simulink model "Resocharge"  (R2023a)
settings: Solver=ode1  StartTime=0.0  StopTime=.4  FixedStep=2e-7  RelTol=1e-3
undefined symbols (not defined in the file): Ion, Lithium
libraries: spsSeriesRLCBranchLib x6, spsVoltageMeasurementLib x6, spsCurrentMeasurementLib x5, spsDiodeLib x4, spsMosfetLib x4, spsACVoltageSourceLib x1, spsBatteryLib x1, simulink x1, spsMutualInductanceLib x1, spsUniversalBridgeLib x1, spspowerguiLib x1
settings Model: Creator=Harish Kumar M  LastModifiedBy=Harish Kumar M

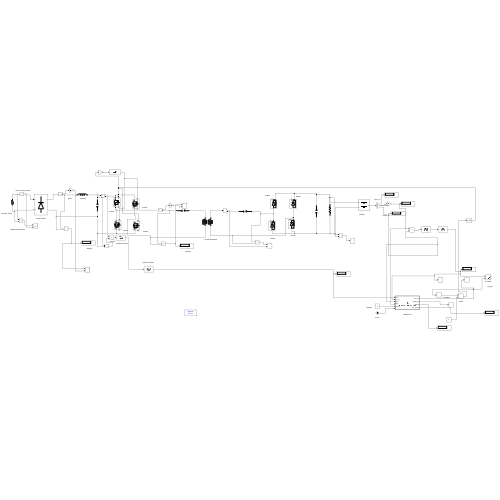
[thumbnail: Simulink's stored preview of the top-level diagram]
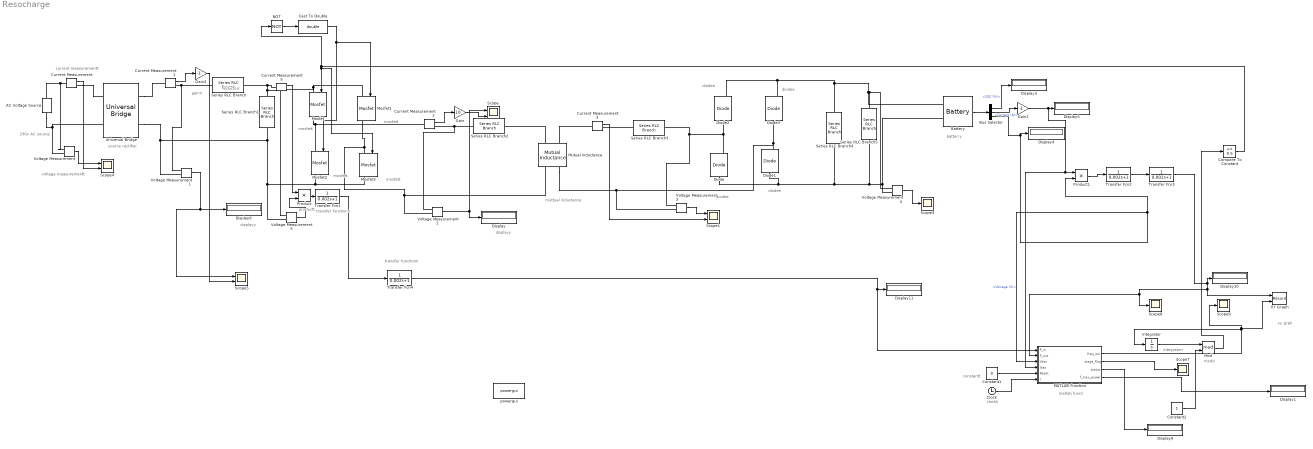
== system Resocharge ==
  note: modd
  note: xy grph
  note: integratorr
  note: constantt
  note: clockk
  note: matlab funcn
  note: batterry
  note: displayy
  note: diodee
  note: muttual inductance
  note: productt
  note: transfer functionn
  note: mosfett
  note: inductorr
  note: gainn
  note: source rectifier
  note: voltage measurementt
  note: 230v AC source
  note: current measurementt
  note: transfer functionn
  note: diodee
  note: diodee
  note: diodee
  note: mosfett
  note: mosfett
  note: mosfett
  note: displayy
  AC Voltage Source : spsACVoltageSourceLib/AC Voltage Source  Amplitude=230*sqrt(2)  Phase=0  Frequency=50  SampleTime=0  Measurements=None  BusType=swing  Pref=10e3  Qref=0  Qmin=-inf  Qmax=+inf
  Battery : spsBatteryLib/Battery  BatType=Lithium-Ion  ShowTempParam=off  ThermalPreset=no  ShowAgeParam=off  NomV=400  NomQ=100  SOC=50  Batt_Tr=1  PresetModel=on  MaxQ=100  MinV=300  FullV=465.5949  Dis_rate=43.4783  R=0.04  Normal_OP=90.4348  expZone="[432.1543      4.913043]"  current=[6.5 13 32.5]  Units=Time  Tci=20  NomT=20  T2=-30  MaxQ2=4.8  FullV2=7.1  Normal_OP2=5.655  expZone2="[6.58           1]"  Rca=0.6  ti=2000  Dp=0  Neq0=0  Tsim=1e6  Ta1=25  Qeol=5.4*0.9  Reol=0.013333*1.2  Char_age=[2.3478, 3]  Dis_age=[2.3478, 10]  N1=1500  N2=10500  N3=1000  N4=1400  Ta2=45  N5=950
  Bus Selector : BusSelector  OutputSignals=SOC (%),Current (A),Voltage (V)
  Cast To Double : DataTypeConversion  OutDataTypeStr=double  SaturateOnIntegerOverflow=off  RndMeth=Floor
  Clock : Clock
  Compare To Constant : simulink/Logic and Bit Operations/Compare To Constant  relop=<=  const=0.5  OutDataTypeStr=boolean
  Constant1 : Constant  Value=0
  Constant2 : Constant
  Current Measurement{,1..3,5} (5 alike) : spsCurrentMeasurementLib/Current Measurement  PhasorSimulation=off  OutputType=Complex  PSBequivalent=0
  Diode{,1..3} (4 alike) : spsDiodeLib/Diode  Ron=0.001  Lon=0  Vf=0.8  IC=0  UseSnubber=0  Rs=500  Cs=250e-9  Measurements=on
  Display{,1,3..6,9..11} (9 alike) : Display
  Gain : Gain  Gain=10
  Gain2 : Gain  Gain=-1
  Gain3 : Gain  Gain=-1
  Integrator : Integrator
  MATLAB Function : MATLAB Function  TreatAsAtomicUnit=on  SystemSampleTime=1e-4
  Mod : Math  Operator=mod
  Mosfet{,1..3} (4 alike) : spsMosfetLib/Mosfet  Ron=0.1  Lon=0  Rd=0.01  Vfd=0  IC=0  Rs=1e5  Cs=inf  Measurements=on
  Mutual Inductance : spsMutualInductanceLib/Mutual Inductance  LConnTagsString=a|b  RConnTagsString=A|B  TypeOfMutual=Two or three windings with equal mutual terms  NumberOfWindings=3  SelfImpedance1=[0.05 110e-06]  SelfImpedance2=[ 0.05 110e-6]  ThreeWindings=off  SelfImpedance3=[ 1.1 1.1e-03]  MutualImpedance=[0 27.5e-06]  InductanceMatrix="[1.0 0.9  0.9 ;  0.9 1.0  0.9;  0.9 0.9 1.0 ] * 1e-3"  ResistanceMatrix="[1.0 0.9  0.9 ;  0.9 1.0  0.9;  0.9 0.9 1.0 ]"  Measurements=None
      settings: LibrarySourceBlock=sps_lib/Passives/Mutual Inductance
  NOT : Logic  Operator=NOT  IconShape=distinctive  AllPortsSameDT=off  OutDataTypeStr=boolean
  Product : Product
  Product1 : Product
  Scope{,1,4..5} (4 alike) : Scope  NumInputPorts=2
  Scope{3,7..9} (4 alike) : Scope
  Series RLC Branch : spsSeriesRLCBranchLib/Series RLC Branch  LConnTagsString=__new0  RConnTagsString=__new0  BranchType=L  Resistance=1  Inductance=5e-3  SetiL0=off  InitialCurrent=0  Capacitance=1e-6  Setx0=off  InitialVoltage=0  Measurements=None
  Series RLC Branch1 : spsSeriesRLCBranchLib/Series RLC Branch  LConnTagsString=__new0  RConnTagsString=__new0  BranchType=C  Resistance=1  Inductance=1e-3  SetiL0=off  InitialCurrent=0  Capacitance=3300e-6  Setx0=off  InitialVoltage=0  Measurements=None
  Series RLC Branch2 : spsSeriesRLCBranchLib/Series RLC Branch  LConnTagsString=__new0  RConnTagsString=__new0  BranchType=C  Resistance=1  Inductance=1e-3  SetiL0=off  InitialCurrent=0  Capacitance=38.8e-9  Setx0=off  InitialVoltage=0  Measurements=None
  Series RLC Branch3 : spsSeriesRLCBranchLib/Series RLC Branch  LConnTagsString=__new0  RConnTagsString=__new0  BranchType=C  Resistance=1  Inductance=1e-3  SetiL0=off  InitialCurrent=0  Capacitance=38.8e-9  Setx0=off  InitialVoltage=0  Measurements=None
  Series RLC Branch4 : spsSeriesRLCBranchLib/Series RLC Branch  LConnTagsString=__new0  RConnTagsString=__new0  BranchType=C  Resistance=1  Inductance=1e-3  SetiL0=off  InitialCurrent=0  Capacitance=100e-6  Setx0=on  InitialVoltage=325  Measurements=None
  Series RLC Branch5 : spsSeriesRLCBranchLib/Series RLC Branch  LConnTagsString=__new0  RConnTagsString=__new0  BranchType=R  Resistance=10000  Inductance=1e-3  SetiL0=off  InitialCurrent=0  Capacitance=1e-6  Setx0=off  InitialVoltage=0  Measurements=None
  Transfer Fcn{1..4} (4 alike) : TransferFcn  Denominator=[0.002 1]
  Universal Bridge : spsUniversalBridgeLib/Universal Bridge  Arms=2  SnubberResistance=1e5  SnubberCapacitance=inf  Device=Diodes  Ron=1e-3  Lon=0  ForwardVoltages="[  0  0  ]"  ForwardVoltage=0  GTOparameters=[ 10e-6 , 20e-6 ]  IGBTparameters=[ 1e-6 , 2e-6 ]  Measurements=None  Measurements_2=None  converterType=Rectifier
  Voltage Measurement{,1..5} (6 alike) : spsVoltageMeasurementLib/Voltage Measurement  PhasorSimulation=off  OutputType=Complex  PSBequivalent=0
  XY Graph : Record  FileSettingsInternal="{\"entries\":[{\"content\":{\"excelSettings\":{\"content\":{},\"type\":\"Streamout.ExcelSettings\"}},\"type\":\"Streamout.FileSettingStorage\",\"uuid\":\"\"}],\"packageUris\":[\"http:\\/\\/schema.mathworks.com\\/mf0\\/streamout_blocks\\/R2020a\"],\"version\":\"1.0\"}"  Layout=[1 1]  SignalsInternal="{\"entries\":[{\"content\":{\"signals\":[{\"content\":{\"blockPath\":[],\"dimensions\":[1],\"domain\":\"\",\"lineColor\":\"#a2142f\",\"plots\":[1],\"port\":1,\"signalID\":17,\"signalName\":\"Transfer Fcn3\"},\"type\":\"RecordBlkView.Signal\",\"uuid\":\"\"},{\"content\":{\"blockPath\":[],\"dimensions\":[1],\"domain\":\"\",\"lineColor\":\"#139fff\",\"plots\":[1],\"port\":2,\"signalID\":20,\"signalName\":\"MATLAB Function:1\"},\"type\":\"RecordBlkView.Signal\",\"uuid\":\"\"}]},\"type\":\"RecordBlkView.InputSignals\",\"uuid\":\"\"}],\"packageUris\":[\"http:\\/\\/schema.mathworks.com\\/mf0\\/streamout_blocks\\/R2020a\"],\"version\":\"1.0\"}"  VisualizationBindings="{\"xyplotplugin\":{\"info\":[{\"series\":[{\"bindingParametersList\":[{\"parameter\":\"X-Axis\",\"signalID\":17,\"signalName\":\"Transfer Fcn3\"},{\"parameter\":\"Y-Axis\",\"signalID\":20,\"signalName\":\"MATLAB Function:1\"}],\"seriesID\":38810}],\"subplotID\":1}]}}"  CompatibilityTag=XY
  powergui : spspowerguiLib/powergui  Priority=1  SimulationMode=Discrete  SampleTime=2e-7  frequency=60  Iterations=50  frequencyindice=50  Pbase=100e6  ErrMax=1e-4  UnitsV=kV  UnitsW=MW  buscounter=0  FunctionMessages=off  echomessages=off  EnableUseOfTLC=off  CurrentSourceSwitches=off  DisableSnubberDevices=off  DisableRonSwitches=off  DisableVfSwitches=off  DisplayEquations=off  AutomaticDiscreteSolvers=off  SolverType=Tustin/Backward Euler (TBE)  Interpol=off  ExternalGateDelay=off  methode=off  Ts=100  x0status=blocks  SPID=on  SwTol=0  HookPort=off  NonlinearTolerance=1e-4  nMaxIteration=100  ContinueOnMaxIteration=off  RestoreLinks=warning  ResistiveCurrentMeasurement=off  Frange=[0:2:500]  Ylog=off  Xlog=on  ShowGrid=off  save=off  variable=ZData  structure=0  ZoomFFT=off  StartTime=0.0  cycles=1  DisplayStyle=1  fundamental=60  FreqAxis=off  MaxFrequency=1000  frequencyindicesteady=1  RmsSteady=1  display=off
  wires:
  NOT/1 -> Cast To Double/1
  Cast To Double/1 -> Mosfet1/1, Mosfet2/1
  Current Measurement2/1 -> Gain/1
  Voltage Measurement2/1 -> Scope/1, Display/1
  Current Measurement3/1 -> Scope1/2
  Voltage Measurement3/1 -> Scope1/1
  Voltage Measurement4/1 -> Scope3/1
  Battery/1 -> Bus Selector/1
  Bus Selector/1 -> Display3/1  "<SOC (%)>"
  Bus Selector/3 -> Product1/2, MATLAB Function/3(Vbat), Display4/1  "<Voltage (V)>"
  Bus Selector/2 -> Gain2/1  "<Current (A)>"
  Current Measurement/1 -> Scope4/2
  Voltage Measurement/1 -> Scope4/1
  Current Measurement1/1 -> Gain3/1
  Gain3/1 -> Scope5/2
  Voltage Measurement1/1 -> Display6/1, Scope5/1
  Gain/1 -> Scope/2
  Current Measurement5/1 -> Product/1
  Voltage Measurement5/1 -> Product/2
  Product/1 -> Transfer Fcn1/1
  Transfer Fcn1/1 -> Transfer Fcn4/1
  Product1/1 -> Transfer Fcn2/1
  Integrator/1 -> Mod/1
  Constant2/1 -> Mod/2
  Mod/1 -> Compare To Constant/1
  Compare To Constant/1 -> NOT/1, Mosfet3/1, Mosfet/1
  MATLAB Function/2(stage_flag) -> Scope7/1
  Transfer Fcn2/1 -> Transfer Fcn3/1
  Transfer Fcn3/1 -> Display10/1, XY Graph/1, MATLAB Function/2(P_out), Scope8/1
  Transfer Fcn4/1 -> MATLAB Function/1(P_in), Display11/1
  MATLAB Function/3(status) -> Display9/1
  Constant1/1 -> MATLAB Function/5(Reset)
  Clock/1 -> MATLAB Function/6(t)
  Gain2/1 -> MATLAB Function/4(Ibat), Product1/1, Display5/1
  MATLAB Function/1(freq_out) -> Integrator/1, XY Graph/2, Scope9/1
  MATLAB Function/4(f_max_power) -> Display1/1
  connections:
  AC Voltage Source/RConn1 -- Voltage Measurement/LConn1 -- Current Measurement/LConn1
  AC Voltage Source/LConn1 -- Voltage Measurement/LConn2 -- Universal Bridge/LConn2
  Current Measurement/RConn1 -- Universal Bridge/LConn1
  Universal Bridge/RConn1 -- Current Measurement1/LConn1
  Universal Bridge/RConn2 -- Voltage Measurement1/LConn2 -- Series RLC Branch1/RConn1 -- Voltage Measurement5/LConn2 -- Mosfet3/RConn1 -- Mosfet2/RConn1
  Series RLC Branch/LConn1 -- Voltage Measurement1/LConn1 -- Current Measurement1/RConn1
  Mosfet1/LConn1 -- Current Measurement5/RConn1 -- Mosfet/LConn1
  Mosfet2/LConn1 -- Current Measurement2/LConn1 -- Mosfet/RConn1
  Series RLC Branch2/LConn1 -- Voltage Measurement2/LConn1 -- Current Measurement2/RConn1
  Mutual Inductance/LConn1 -- Series RLC Branch2/RConn1
  Mosfet3/LConn1 -- Voltage Measurement2/LConn2 -- Mutual Inductance/RConn1 -- Mosfet1/RConn1
  Mutual Inductance/LConn2 -- Current Measurement3/LConn1
  Series RLC Branch3/LConn1 -- Current Measurement3/RConn1
  Diode1/RConn1 -- Voltage Measurement3/LConn2 -- Mutual Inductance/RConn2 -- Diode3/LConn1
  Diode/LConn1 -- Battery/LConn2 -- Voltage Measurement4/LConn2 -- Series RLC Branch5/RConn1 -- Series RLC Branch4/RConn1 -- Diode1/LConn1
  Voltage Measurement3/LConn1 -- Diode/RConn1 -- Diode2/LConn1 -- Series RLC Branch3/RConn1
  Diode2/RConn1 -- Series RLC Branch4/LConn1 -- Series RLC Branch5/LConn1 -- Voltage Measurement4/LConn1 -- Battery/LConn1 -- Diode3/RConn1
  Series RLC Branch1/LConn1 -- Voltage Measurement5/LConn1 -- Series RLC Branch/RConn1 -- Current Measurement5/LConn1

== matlab function Resocharge/MATLAB Function ==
  data: freq_out output; stage_flag output; status output; P_in input; P_out input; Vbat input; Ibat input; Reset input; t input; f_max_power output
function [freq_out, stage_flag, status, f_max_power] = Adaptive_Freq_Controller(P_in, P_out, Vbat, Ibat, Reset, t)
% =========================================================================
% TWO-STAGE SEARCH CONTROLLER  |  80 kHz - 90 kHz  |  TARGET 8.25 A
% Hardware assumption: Cp = Cs = 38.8 nF  ->  resonance = 77 kHz
% Therefore inside 80-90 kHz:  FREQ UP = CURRENT DOWN
% =========================================================================

    I_target = 8.25;      % target charging current [A]
    V_max    = 450;       % battery voltage limit [V]
    f_min    = 80000;     % hard lower bound [Hz]
    f_max    = 90000;     % hard upper bound [Hz]
    f_step   = 500;       % staircase step [Hz]
    t_settle = 0.01;      % 10 ms per stair -> 20 stairs -> 0.20 s sweep

    persistent f_current stage f_best I_best_err t_last;

    % ---- Initialisation ----
    if isempty(f_current) || Reset > 0.5
        f_current  = f_min;     % staircase always starts at 80 kHz
        stage      = 1;
        f_best     = f_min;
        I_best_err = 999;
        t_last     = 0;
    end

    % ---- Input cleaning ----
    if isnan(Ibat),  Ibat  = 0; end
    if isnan(Vbat),  Vbat  = 0; end
    if isnan(P_out), P_out = 0; end

    % ---- Execution every 10 ms ----
    if (t - t_last) >= t_settle
        t_last = t;

        if stage == 1
            % ================= STAGE 1 : RISING STAIRCASE =================
            % Record the stair whose current is closest to 8.25 A
            if (t > 0.02) && (Vbat <= V_max)
                err = abs(Ibat - I_target);
                if err < I_best_err
                    I_best_err = err;
                    f_best     = f_current;
                end
            end

            if f_current < f_max
                f_current = f_current + f_step;      % visible staircase
            else
                stage     = 2;
                f_current = f_best;                  % jump to best stair
            end

        else
            % ================= STAGE 2 : FINE LOCK AT 8.25 A =================
            I_err = I_target - Ibat;        % +ve = current too LOW

            % Deadband: freeze when within +/- 0.03 A
            if abs(I_err) <= 0.03
                I_err = 0;
            end

            % *** CORRECT DIRECTION FOR 38.8 nF (resonance below 80 kHz) ***
            % Current too LOW  -> move frequency DOWN toward 77 kHz peak
            % Current too HIGH -> move frequency UP away from peak
            f_delta = -30 * I_err;

            % Adaptive clamp: big moves far away, tiny moves when close
            if abs(I_err) > 1.0
                f_delta = max(min(f_delta, 250), -250);
            else
                f_delta = max(min(f_delta, 60), -60);
            end

            % Voltage protection override
            if Vbat > V_max
                f_delta = 250;              % push up, cut power
            end

            f_current = max(min(f_current + f_delta, f_max), f_min);
        end
    end

    % ---- Outputs ----
    freq_out    = f_current;
    stage_flag  = stage;
    f_max_power = f_best;

    if (Vbat > V_max) || (Ibat > I_target + 0.3)
        status = 1;                         % limit active
    elseif (stage == 2) && (Ibat < I_target - 0.5)
        status = 2;                         % cannot reach target (weak coupling)
    else
        status = 0;                         % normal / locked
    end
end
